simulink model "cll_zcs_ver_v"  (R2026b)
settings: Solver=ode23tb  StopTime=simlength  FixedStep=tc  MaxStep=tc  EnableMultiTasking=on
PostLoadFcn:
  | if any(exist('dsrtsu_mdlpostloadfcn', 'file') ~= 0), dsrtsu_mdlpostloadfcn('Execute', bdroot); end
InitFcn:
  | , if any(exist('rtifpga_mdlclblib', 'file') ~= 0), rtifpga_mdlclblib('Init', bdroot); end,
  | , if any(exist('dsmpb_private', 'file') ~= 0), dsmpb_private('dsmpb_mdlclblib', 'Init', bdroot); end,
values from neighbouring files (symbols this model uses):
  Adrso = eye(2) + Arso*ts    [init_zcs_model_ctrl.m]
  Adrsoh = eye(2) + Arsoh*ts    [init_zcs_model_ctrl.m]
  Crso = [1 0]    [init_zcs_model_ctrl.m]
  Crsoh = [1 0]    [init_zcs_model_ctrl.m]
  fres = 1/2/pi/sqrt(Cs*(Ls+L1sigma))    [init_zcs_model_ctrl.m]
  I_FS = Iout_dc_nom * margin_factor    (= 125)    [init_zcs_model_ctrl.m]
  Iout_ref_SI = 100*scale    (= 100)    [init_zcs_model_ctrl.m]
  k_h10_comp = -12    [init_zcs_model_ctrl.m]
  k_h12_comp = -12    [init_zcs_model_ctrl.m]
  k_h14_comp = -12    [init_zcs_model_ctrl.m]
  k_h2_comp = -12    [init_zcs_model_ctrl.m]
  k_h4_comp = -12    [init_zcs_model_ctrl.m]
  k_h6_comp = -12    [init_zcs_model_ctrl.m]
  k_h8_comp = -12    [init_zcs_model_ctrl.m]
  ki_i_zcs = 80    [init_zcs_model_ctrl.m]
  ki_v_zcs = 80    [init_zcs_model_ctrl.m]
  kp_i_zcs = 0.25    [init_zcs_model_ctrl.m]
  kp_v_zcs = 0.25    [init_zcs_model_ctrl.m]
  Ldrso = acker(Adrso',Crso',polesdrso)'    [init_zcs_model_ctrl.m]
  Ldrsoh = acker(Adrsoh',Crsoh',polesdrsoh)'    [init_zcs_model_ctrl.m]
  omega_grid_emu_nom = w_grid    (= 314.159265359)    [grid_emulator.m]
  omega_grid_nom = w_grid    (= 314.159265359)    [grid_emulator.m]
  pll_i1 = 80    [init_zcs_model_ctrl.m]
  pll_p = 1    [init_zcs_model_ctrl.m]
  q1kalman = ts/10    (= 1e-05)    [init_zcs_model_ctrl.m]
  q2kalman = ts/10    (= 1e-05)    [init_zcs_model_ctrl.m]
  Rkalman = 1/ts    (= 10000)    [init_zcs_model_ctrl.m]
  tc = 1e-7    (= 1e-07)    [init_zcs_model_ctrl.m]
  ts = 1e-4    (= 0.0001)    [init_zcs_model_ctrl.m]
  V_FS = Vout_dc_nom * margin_factor    (= 12.5)    [init_zcs_model_ctrl.m]
  V_phase_normalization_factor = Vgrid_phase_normalization_factor    [grid_emulator.m]
  Vgrid_phase_normalization_factor = Vphase2*sqrt(2)    [grid_emulator.m]
  vn_eta_pu = 0.05    [init_zcs_model_ctrl.m]
  vn_xi_pu = 0.05    [init_zcs_model_ctrl.m]
  Vout_dc_nom = 10    [init_zcs_model_ctrl.m]
  vp_xi_pu = 0.9    [init_zcs_model_ctrl.m]
undefined symbols (not defined in the file or in its folder): magnitude
libraries: fl_lib x55, nesl_utility x18, cstblocks_lti x7, single_phase_transformer_lib x1
(part 2 of 2)

== system cll_zcs_ver_v/vi_ctrl/sampling_v_filter1 ==
  in : Inport
  1/Ti3 : Gain  Gain=1/V_FS  OutDataTypeStr=double  SaturateOnIntegerOverflow=on  ParamDataTypeStr=Inherit: Same as input
  Saturation : Saturate  UpperLimit=1  LowerLimit=0  OutDataTypeStr=double
  Zero-Order Hold2 : ZeroOrderHold  SampleTime=ts
  out_pu : Outport
  wires:
  Zero-Order Hold2/1 -> out_pu/1
  1/Ti3/1 -> Saturation/1
  in/1 -> 1/Ti3/1
  Saturation/1 -> Zero-Order Hold2/1

== system cll_zcs_ver_v/vi_ctrl/sampling_v_filter2 ==
  in : Inport
  1/Ti3 : Gain  Gain=1/V_FS  OutDataTypeStr=double  SaturateOnIntegerOverflow=on  ParamDataTypeStr=Inherit: Same as input
  Saturation : Saturate  UpperLimit=1  LowerLimit=0  OutDataTypeStr=double
  Zero-Order Hold2 : ZeroOrderHold  SampleTime=ts
  out_pu : Outport
  wires:
  in/1 -> 1/Ti3/1
  1/Ti3/1 -> Saturation/1
  Zero-Order Hold2/1 -> out_pu/1
  Saturation/1 -> Zero-Order Hold2/1

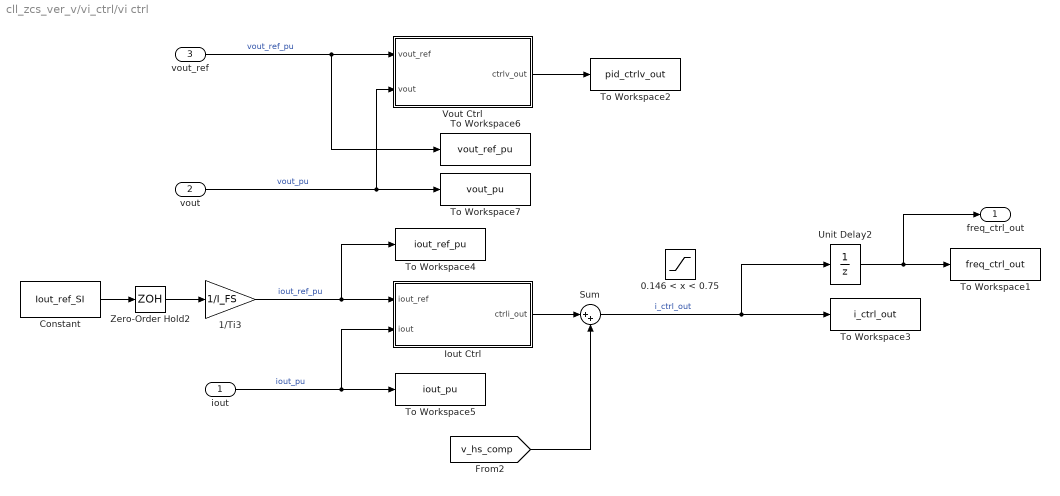
== system cll_zcs_ver_v/vi_ctrl/vi ctrl ==
  iout : Inport
  vout : Inport  Port=2
  vout_ref : Inport  Port=3
  0.146 < x < 0.75 : Saturate  UpperLimit=0.75  LowerLimit=0.146  OutDataTypeStr=double
  1/Ti3 : Gain  Gain=1/I_FS  OutDataTypeStr=double  SaturateOnIntegerOverflow=on  ParamDataTypeStr=Inherit: Same as input
  Constant : Constant  Value=Iout_ref_SI
  Iout Ctrl : Subsystem
  Sum : Sum  Inputs=|++
  To Workspace1 : ToWorkspace  VariableName=freq_ctrl_out  SampleTime=ts
      settings: MaxDataPoints=Ns
  To Workspace2 : ToWorkspace  VariableName=pid_ctrlv_out  SampleTime=ts
      settings: MaxDataPoints=Ns  Save2DSignal=2-D array (concatenate along first dimension)
  To Workspace3 : ToWorkspace  VariableName=i_ctrl_out  SampleTime=ts
      settings: MaxDataPoints=Ns  Save2DSignal=2-D array (concatenate along first dimension)
  To Workspace4 : ToWorkspace  VariableName=iout_ref_pu  SampleTime=ts
      settings: MaxDataPoints=Ns  Save2DSignal=2-D array (concatenate along first dimension)
  To Workspace5 : ToWorkspace  VariableName=iout_pu  SampleTime=ts
      settings: MaxDataPoints=Ns  Save2DSignal=2-D array (concatenate along first dimension)
  To Workspace6 : ToWorkspace  VariableName=vout_ref_pu  SampleTime=ts
      settings: MaxDataPoints=Ns  Save2DSignal=2-D array (concatenate along first dimension)
  To Workspace7 : ToWorkspace  VariableName=vout_pu  SampleTime=ts
      settings: MaxDataPoints=Ns  Save2DSignal=2-D array (concatenate along first dimension)
  Unit Delay2 : UnitDelay  SampleTime=ts
  Vout Ctrl : Subsystem
  Zero-Order Hold2 : ZeroOrderHold  SampleTime=ts
  freq_ctrl_out : Outport
  wires:
  Unit Delay2/1 -> To Workspace1/1, freq_ctrl_out/1
  iout/1 -> To Workspace5/1, Iout Ctrl/2(iout)  "iout_pu"
  vout_ref/1 -> To Workspace6/1, Vout Ctrl/1(vout_ref)  "vout_ref_pu"
  vout/1 -> Vout Ctrl/2(vout), To Workspace7/1  "vout_pu"
  Vout Ctrl/1(ctrlv_out) -> To Workspace2/1
  Constant/1 -> Zero-Order Hold2/1
  1/Ti3/1 -> To Workspace4/1, Iout Ctrl/1(iout_ref)  "iout_ref_pu"
  Iout Ctrl/1(ctrli_out) -> Sum/1
  Zero-Order Hold2/1 -> 1/Ti3/1
  Sum/1 -> Unit Delay2/1, To Workspace3/1  "i_ctrl_out"
  [v_hs_comp] -> Sum/2

== system cll_zcs_ver_v/PLL/pll_stageA/mormalization_and_transformation ==
  ug_a : Inport
  ug_b : Inport  Port=2
  ug_c : Inport  Port=3
  Gain1 : Gain  Gain=1/Vgrid_phase_normalization_factor
  Gain2 : Gain  Gain=1/Vgrid_phase_normalization_factor
  Gain3 : Gain  Gain=1/Vgrid_phase_normalization_factor
  Zero-Order Hold : ZeroOrderHold  SampleTime=ts
  Zero-Order Hold1 : ZeroOrderHold  SampleTime=ts
  Zero-Order Hold2 : ZeroOrderHold  SampleTime=ts
  abc2alphabeta : MATLAB Function  TreatAsAtomicUnit=on
  ug_alpha : Outport  VectorParamsAs1DForOutWhenUnconnected=off
  ug_beta : Outport  Port=2  VectorParamsAs1DForOutWhenUnconnected=off
  wires:
  abc2alphabeta/1(alpha) -> ug_alpha/1  "u_grid_alpha"
  abc2alphabeta/2(beta) -> ug_beta/1  "u_grid_beta"
  Gain3/1 -> abc2alphabeta/3(c)
  Gain2/1 -> abc2alphabeta/2(b)
  Gain1/1 -> abc2alphabeta/1(a)
  Zero-Order Hold2/1 -> Gain3/1
  Zero-Order Hold1/1 -> Gain2/1
  Zero-Order Hold/1 -> Gain1/1
  ug_b/1 -> Zero-Order Hold1/1
  ug_c/1 -> Zero-Order Hold2/1
  ug_a/1 -> Zero-Order Hold/1

== system cll_zcs_ver_v/PLL/pll_stageA/sequences ==
  u_grid_alpha : Inport
  u_grid_beta : Inport  Port=2
  phase_angle : Inport  Port=3
  ddsrf : Subsystem
  u_grid_pos_xi : Outport
  u_grid_pos_eta : Outport  Port=2
  wires:
  phase_angle/1 -> ddsrf/3(phase_angle)  "phase_angle"
  u_grid_beta/1 -> ddsrf/2(u_grid_beta)  "u_grid_beta"
  u_grid_alpha/1 -> ddsrf/1(u_grid_alpha)  "u_grid_alpha"
  ddsrf/2(u_grid_pos_eta) -> u_grid_pos_eta/1  "u_grid_pos_eta"
  ddsrf/1(u_grid_pos_xi) -> u_grid_pos_xi/1  "u_grid_pos_xi"

== system cll_zcs_ver_v/PLL/pll_stageB/double_integrator_observer ==
  theta : Inport
  Gain : Gain  Gain=Ldrso  Multiplication=Matrix(K*u)
  Gain1 : Gain  Gain=Adrso  Multiplication=Matrix(K*u)
  Gain2 : Gain  Gain=Crso  Multiplication=Matrix(K*u)
  Selector : Selector  InputPortWidth=2  IndexOptions=Index vector (dialog)  Indices=2  OutputSizes=1  RuntimeRangeChecks=off
  Sum : Sum  Inputs=-+|
  Sum1 : Sum  Inputs=|++
  Unit Delay : UnitDelay  SampleTime=ts
  Zero-Order Hold : ZeroOrderHold  SampleTime=ts
  bounder1 : MATLAB Function  TreatAsAtomicUnit=on  SystemSampleTime=ts
  bounder2 : MATLAB Function  TreatAsAtomicUnit=on  SystemSampleTime=ts
  omega_hat : Outport
  wires:
  bounder2/1(y) -> Sum/1  "theta_hat_bounded"
  bounder1/1(y) -> Gain/1  "e_bounded"
  Zero-Order Hold/1 -> Sum/2  "theta_dsp"
  theta/1 -> Zero-Order Hold/1  "theta"
  Unit Delay/1 -> Gain2/1, Selector/1, Gain1/1
  Sum/1 -> bounder1/1(u)  "e"
  Sum1/1 -> Unit Delay/1
  Gain1/1 -> Sum1/2
  Gain2/1 -> bounder2/1(u)  "theta_hat"
  Selector/1 -> omega_hat/1
  Gain/1 -> Sum1/1

== system cll_zcs_ver_v/cll_zcs/HBridge/switch_1 ==
  g : Inport
  D : fl_lib/Electrical/Electrical Elements/Diode  Vf=0.6 V  Ron=1e-3 Ohm  Goff=1e-8 1/Ohm  i_specify=off  i_priority=None  i=0 A  i_nominal_specify=off  i_nominal_value=1  i_nominal_unit=A  v_specify=off  v_priority=None  v=0 V  v_nominal_specify=off  v_nominal_value=1  v_nominal_unit=V
  Q : fl_lib/Electrical/Electrical Elements/Switch  R_closed=1e-3 Ohm  G_open=1e-8 1/Ohm  Threshold=0.5  i_specify=off  i_priority=None  i=0 A  i_nominal_specify=off  i_nominal_value=1  i_nominal_unit=A  v_specify=off  v_priority=None  v=0 V  v_nominal_specify=off  v_nominal_value=1  v_nominal_unit=V
  RCsnubber : fl_lib/Electrical/Electrical Elements/Capacitor  c=Csnubber F  r=Rsnubber Ohm  g=0 1/Ohm  i_specify=off  i_priority=None  i=0 A  i_nominal_specify=off  i_nominal_value=1  i_nominal_unit=A  v_specify=off  v_priority=None  v=0 V  v_nominal_specify=off  v_nominal_value=1  v_nominal_unit=V  vc_specify=off  vc_priority=High  vc=0 V  vc_nominal_specify=off  vc_nominal_value=1  vc_nominal_unit=V
  Simulink-PS Converter : nesl_utility/Simulink-PS Converter  PhysicalDomain=network_engine_domain  SubClassName=ps_input  LeftPortType=input  RightPortType=output  PseudoPeriodic=off  Frequencies=[]  NoiseDistribution=none  NoiseParameters=[]  Unit=1  AffineConversion=off  FilteringAndDerivatives=provide  SimscapeFilterOrder=1  InputFilterTimeConstant=0.001  UdotUserProvided=0
  d : PMIOPort  Side=Left
  s : PMIOPort  Port=2  Side=Right
  wires:
  g/1 -> Simulink-PS Converter/1
  connections:
  Q/RConn2 -- D/LConn1 -- s/RConn1 -- RCsnubber/RConn1
  Simulink-PS Converter/RConn1 -- Q/RConn1
  Q/LConn1 -- RCsnubber/LConn1 -- d/RConn1 -- D/RConn1

== system cll_zcs_ver_v/cll_zcs/HBridge/switch_2 ==
  g : Inport
  D : fl_lib/Electrical/Electrical Elements/Diode  Vf=0.6 V  Ron=1e-3 Ohm  Goff=1e-8 1/Ohm  i_specify=off  i_priority=None  i=0 A  i_nominal_specify=off  i_nominal_value=1  i_nominal_unit=A  v_specify=off  v_priority=None  v=0 V  v_nominal_specify=off  v_nominal_value=1  v_nominal_unit=V
  Q : fl_lib/Electrical/Electrical Elements/Switch  R_closed=1e-3 Ohm  G_open=1e-8 1/Ohm  Threshold=0.5  i_specify=off  i_priority=None  i=0 A  i_nominal_specify=off  i_nominal_value=1  i_nominal_unit=A  v_specify=off  v_priority=None  v=0 V  v_nominal_specify=off  v_nominal_value=1  v_nominal_unit=V
  RCsnubber : fl_lib/Electrical/Electrical Elements/Capacitor  c=Csnubber F  r=Rsnubber Ohm  g=0 1/Ohm  i_specify=off  i_priority=None  i=0 A  i_nominal_specify=off  i_nominal_value=1  i_nominal_unit=A  v_specify=off  v_priority=None  v=0 V  v_nominal_specify=off  v_nominal_value=1  v_nominal_unit=V  vc_specify=off  vc_priority=High  vc=0 V  vc_nominal_specify=off  vc_nominal_value=1  vc_nominal_unit=V
  Simulink-PS Converter : nesl_utility/Simulink-PS Converter  PhysicalDomain=network_engine_domain  SubClassName=ps_input  LeftPortType=input  RightPortType=output  PseudoPeriodic=off  Frequencies=[]  NoiseDistribution=none  NoiseParameters=[]  Unit=1  AffineConversion=off  FilteringAndDerivatives=provide  SimscapeFilterOrder=1  InputFilterTimeConstant=0.001  UdotUserProvided=0
  d : PMIOPort  Side=Left
  s : PMIOPort  Port=2  Side=Right
  wires:
  g/1 -> Simulink-PS Converter/1
  connections:
  d/RConn1 -- RCsnubber/LConn1 -- Q/LConn1 -- D/RConn1
  Simulink-PS Converter/RConn1 -- Q/RConn1
  s/RConn1 -- RCsnubber/RConn1 -- D/LConn1 -- Q/RConn2

== system cll_zcs_ver_v/grid/grid_emulator/grid_emulator ==
  phase_gen : Subsystem
  voltage_reference : Subsystem
  voltage_source : Subsystem
  Vma : Outport
  Vmb : Outport  Port=2
  Vmc : Outport  Port=3
  wires:
  phase_gen/1(grid_emu_phase) -> voltage_reference/1(grid_emu_phase)  "grid_emu_phase"
  voltage_source/2(vn_xi) -> voltage_reference/3(Vxi_n)
  voltage_source/1(vp_xi) -> voltage_reference/2(Vxi_p)
  voltage_source/3(vn_eta) -> voltage_reference/4(Veta_n)
  voltage_reference/3(V3_ref) -> Vmc/1
  voltage_reference/1(V1_ref) -> Vma/1
  voltage_reference/2(V2_ref) -> Vmb/1

== system cll_zcs_ver_v/hs_compensation/magnitude_100Hz_harmonic_detection/double_integrator_observer ==
  theta : Inport
  Gain : Gain  Gain=Ldrsoh  Multiplication=Matrix(K*u)
  Gain1 : Gain  Gain=Adrsoh  Multiplication=Matrix(K*u)
  Gain2 : Gain  Gain=Crsoh  Multiplication=Matrix(K*u)
  Selector : Selector  InputPortWidth=2  IndexOptions=Index vector (dialog)  Indices=2  OutputSizes=1  RuntimeRangeChecks=off
  Sum : Sum  Inputs=-+|
  Sum1 : Sum  Inputs=|++
  Unit Delay : UnitDelay  SampleTime=ts
  Zero-Order Hold : ZeroOrderHold  SampleTime=ts
  bounder1 : MATLAB Function  TreatAsAtomicUnit=on  SystemSampleTime=ts
  bounder2 : MATLAB Function  TreatAsAtomicUnit=on  SystemSampleTime=ts
  omega_hat : Outport
  theta_hat : Outport  Port=2
  wires:
  Gain/1 -> Sum1/1
  Selector/1 -> omega_hat/1
  Gain2/1 -> bounder2/1(u)  "theta_hat"
  Gain1/1 -> Sum1/2
  Sum1/1 -> Unit Delay/1
  Sum/1 -> bounder1/1(u)  "e"
  Unit Delay/1 -> Gain1/1, Selector/1, Gain2/1
  theta/1 -> Zero-Order Hold/1  "theta"
  Zero-Order Hold/1 -> Sum/2  "theta_dsp"
  bounder1/1(y) -> Gain/1  "e_bounded"
  bounder2/1(y) -> theta_hat/1, Sum/1  "theta_hat_bounded"

== system cll_zcs_ver_v/hs_compensation/magnitude_100Hz_harmonic_detection/magnitude ==
  alpha : Inport
  beta : Inport  Port=2
  Math Function : Math  Operator=magnitude^2
  Math Function1 : Math  Operator=magnitude^2
  Sqrt : Sqrt
  Sum : Sum  Inputs=|++
  a : Outport
  wires:
  Sqrt/1 -> a/1
  Sum/1 -> Sqrt/1
  Math Function1/1 -> Sum/2
  Math Function/1 -> Sum/1
  beta/1 -> Math Function1/1
  alpha/1 -> Math Function/1

== system cll_zcs_ver_v/hs_compensation/magnitude_200Hz_harmonic_detection/double_integrator_observer ==
  theta : Inport
  Gain : Gain  Gain=Ldrsoh  Multiplication=Matrix(K*u)
  Gain1 : Gain  Gain=Adrsoh  Multiplication=Matrix(K*u)
  Gain2 : Gain  Gain=Crsoh  Multiplication=Matrix(K*u)
  Selector : Selector  InputPortWidth=2  IndexOptions=Index vector (dialog)  Indices=2  OutputSizes=1  RuntimeRangeChecks=off
  Sum : Sum  Inputs=-+|
  Sum1 : Sum  Inputs=|++
  Unit Delay : UnitDelay  SampleTime=ts
  Zero-Order Hold : ZeroOrderHold  SampleTime=ts
  bounder1 : MATLAB Function  TreatAsAtomicUnit=on  SystemSampleTime=ts
  bounder2 : MATLAB Function  TreatAsAtomicUnit=on  SystemSampleTime=ts
  omega_hat : Outport
  theta_hat : Outport  Port=2
  wires:
  Gain/1 -> Sum1/1
  Selector/1 -> omega_hat/1
  Gain2/1 -> bounder2/1(u)  "theta_hat"
  Gain1/1 -> Sum1/2
  Sum1/1 -> Unit Delay/1
  Sum/1 -> bounder1/1(u)  "e"
  Unit Delay/1 -> Gain1/1, Selector/1, Gain2/1
  theta/1 -> Zero-Order Hold/1  "theta"
  Zero-Order Hold/1 -> Sum/2  "theta_dsp"
  bounder1/1(y) -> Gain/1  "e_bounded"
  bounder2/1(y) -> theta_hat/1, Sum/1  "theta_hat_bounded"

== system cll_zcs_ver_v/hs_compensation/magnitude_200Hz_harmonic_detection/magnitude ==
  alpha : Inport
  beta : Inport  Port=2
  Math Function : Math  Operator=magnitude^2
  Math Function1 : Math  Operator=magnitude^2
  Sqrt : Sqrt
  Sum : Sum  Inputs=|++
  a : Outport
  wires:
  alpha/1 -> Math Function/1
  beta/1 -> Math Function1/1
  Math Function/1 -> Sum/1
  Math Function1/1 -> Sum/2
  Sum/1 -> Sqrt/1
  Sqrt/1 -> a/1

== system cll_zcs_ver_v/hs_compensation/magnitude_300Hz_harmonic_detection/double_integrator_observer ==
  theta : Inport
  Gain : Gain  Gain=Ldrsoh  Multiplication=Matrix(K*u)
  Gain1 : Gain  Gain=Adrsoh  Multiplication=Matrix(K*u)
  Gain2 : Gain  Gain=Crsoh  Multiplication=Matrix(K*u)
  Selector : Selector  InputPortWidth=2  IndexOptions=Index vector (dialog)  Indices=2  OutputSizes=1  RuntimeRangeChecks=off
  Sum : Sum  Inputs=-+|
  Sum1 : Sum  Inputs=|++
  Unit Delay : UnitDelay  SampleTime=ts
  Zero-Order Hold : ZeroOrderHold  SampleTime=ts
  bounder1 : MATLAB Function  TreatAsAtomicUnit=on  SystemSampleTime=ts
  bounder2 : MATLAB Function  TreatAsAtomicUnit=on  SystemSampleTime=ts
  omega_hat : Outport
  theta_hat : Outport  Port=2
  wires:
  Gain/1 -> Sum1/1
  Selector/1 -> omega_hat/1
  Gain2/1 -> bounder2/1(u)  "theta_hat"
  Gain1/1 -> Sum1/2
  Sum1/1 -> Unit Delay/1
  Sum/1 -> bounder1/1(u)  "e"
  Unit Delay/1 -> Gain1/1, Selector/1, Gain2/1
  theta/1 -> Zero-Order Hold/1  "theta"
  Zero-Order Hold/1 -> Sum/2  "theta_dsp"
  bounder1/1(y) -> Gain/1  "e_bounded"
  bounder2/1(y) -> theta_hat/1, Sum/1  "theta_hat_bounded"

== system cll_zcs_ver_v/hs_compensation/magnitude_300Hz_harmonic_detection/magnitude ==
  alpha : Inport
  beta : Inport  Port=2
  Math Function : Math  Operator=magnitude^2
  Math Function1 : Math  Operator=magnitude^2
  Sqrt : Sqrt
  Sum : Sum  Inputs=|++
  a : Outport
  wires:
  alpha/1 -> Math Function/1
  beta/1 -> Math Function1/1
  Math Function/1 -> Sum/1
  Math Function1/1 -> Sum/2
  Sum/1 -> Sqrt/1
  Sqrt/1 -> a/1

== system cll_zcs_ver_v/hs_compensation/magnitude_400Hz_harmonic_detection/double_integrator_observer ==
  theta : Inport
  Gain : Gain  Gain=Ldrsoh  Multiplication=Matrix(K*u)
  Gain1 : Gain  Gain=Adrsoh  Multiplication=Matrix(K*u)
  Gain2 : Gain  Gain=Crsoh  Multiplication=Matrix(K*u)
  Selector : Selector  InputPortWidth=2  IndexOptions=Index vector (dialog)  Indices=2  OutputSizes=1  RuntimeRangeChecks=off
  Sum : Sum  Inputs=-+|
  Sum1 : Sum  Inputs=|++
  Unit Delay : UnitDelay  SampleTime=ts
  Zero-Order Hold : ZeroOrderHold  SampleTime=ts
  bounder1 : MATLAB Function  TreatAsAtomicUnit=on  SystemSampleTime=ts
  bounder2 : MATLAB Function  TreatAsAtomicUnit=on  SystemSampleTime=ts
  omega_hat : Outport
  theta_hat : Outport  Port=2
  wires:
  Gain/1 -> Sum1/1
  Selector/1 -> omega_hat/1
  Gain2/1 -> bounder2/1(u)  "theta_hat"
  Gain1/1 -> Sum1/2
  Sum1/1 -> Unit Delay/1
  Sum/1 -> bounder1/1(u)  "e"
  Unit Delay/1 -> Gain1/1, Selector/1, Gain2/1
  theta/1 -> Zero-Order Hold/1  "theta"
  Zero-Order Hold/1 -> Sum/2  "theta_dsp"
  bounder1/1(y) -> Gain/1  "e_bounded"
  bounder2/1(y) -> theta_hat/1, Sum/1  "theta_hat_bounded"

== system cll_zcs_ver_v/hs_compensation/magnitude_400Hz_harmonic_detection/magnitude ==
  alpha : Inport
  beta : Inport  Port=2
  Math Function : Math  Operator=magnitude^2
  Math Function1 : Math  Operator=magnitude^2
  Sqrt : Sqrt
  Sum : Sum  Inputs=|++
  a : Outport
  wires:
  alpha/1 -> Math Function/1
  beta/1 -> Math Function1/1
  Math Function/1 -> Sum/1
  Math Function1/1 -> Sum/2
  Sum/1 -> Sqrt/1
  Sqrt/1 -> a/1

== system cll_zcs_ver_v/hs_compensation/magnitude_500Hz_harmonic_detection/double_integrator_observer ==
  theta : Inport
  Gain : Gain  Gain=Ldrsoh  Multiplication=Matrix(K*u)
  Gain1 : Gain  Gain=Adrsoh  Multiplication=Matrix(K*u)
  Gain2 : Gain  Gain=Crsoh  Multiplication=Matrix(K*u)
  Selector : Selector  InputPortWidth=2  IndexOptions=Index vector (dialog)  Indices=2  OutputSizes=1  RuntimeRangeChecks=off
  Sum : Sum  Inputs=-+|
  Sum1 : Sum  Inputs=|++
  Unit Delay : UnitDelay  SampleTime=ts
  Zero-Order Hold : ZeroOrderHold  SampleTime=ts
  bounder1 : MATLAB Function  TreatAsAtomicUnit=on  SystemSampleTime=ts
  bounder2 : MATLAB Function  TreatAsAtomicUnit=on  SystemSampleTime=ts
  omega_hat : Outport
  theta_hat : Outport  Port=2
  wires:
  Gain/1 -> Sum1/1
  Selector/1 -> omega_hat/1
  Gain2/1 -> bounder2/1(u)  "theta_hat"
  Gain1/1 -> Sum1/2
  Sum1/1 -> Unit Delay/1
  Sum/1 -> bounder1/1(u)  "e"
  Unit Delay/1 -> Gain1/1, Selector/1, Gain2/1
  theta/1 -> Zero-Order Hold/1  "theta"
  Zero-Order Hold/1 -> Sum/2  "theta_dsp"
  bounder1/1(y) -> Gain/1  "e_bounded"
  bounder2/1(y) -> theta_hat/1, Sum/1  "theta_hat_bounded"

== system cll_zcs_ver_v/hs_compensation/magnitude_500Hz_harmonic_detection/magnitude ==
  alpha : Inport
  beta : Inport  Port=2
  Math Function : Math  Operator=magnitude^2
  Math Function1 : Math  Operator=magnitude^2
  Sqrt : Sqrt
  Sum : Sum  Inputs=|++
  a : Outport
  wires:
  Sqrt/1 -> a/1
  Sum/1 -> Sqrt/1
  Math Function1/1 -> Sum/2
  Math Function/1 -> Sum/1
  beta/1 -> Math Function1/1
  alpha/1 -> Math Function/1

== system cll_zcs_ver_v/hs_compensation/magnitude_600Hz_harmonic_detection/double_integrator_observer ==
  theta : Inport
  Gain : Gain  Gain=Ldrsoh  Multiplication=Matrix(K*u)
  Gain1 : Gain  Gain=Adrsoh  Multiplication=Matrix(K*u)
  Gain2 : Gain  Gain=Crsoh  Multiplication=Matrix(K*u)
  Selector : Selector  InputPortWidth=2  IndexOptions=Index vector (dialog)  Indices=2  OutputSizes=1  RuntimeRangeChecks=off
  Sum : Sum  Inputs=-+|
  Sum1 : Sum  Inputs=|++
  Unit Delay : UnitDelay  SampleTime=ts
  Zero-Order Hold : ZeroOrderHold  SampleTime=ts
  bounder1 : MATLAB Function  TreatAsAtomicUnit=on  SystemSampleTime=ts
  bounder2 : MATLAB Function  TreatAsAtomicUnit=on  SystemSampleTime=ts
  omega_hat : Outport
  theta_hat : Outport  Port=2
  wires:
  Gain/1 -> Sum1/1
  Selector/1 -> omega_hat/1
  Gain2/1 -> bounder2/1(u)  "theta_hat"
  Gain1/1 -> Sum1/2
  Sum1/1 -> Unit Delay/1
  Sum/1 -> bounder1/1(u)  "e"
  Unit Delay/1 -> Gain1/1, Selector/1, Gain2/1
  theta/1 -> Zero-Order Hold/1  "theta"
  Zero-Order Hold/1 -> Sum/2  "theta_dsp"
  bounder1/1(y) -> Gain/1  "e_bounded"
  bounder2/1(y) -> theta_hat/1, Sum/1  "theta_hat_bounded"

== system cll_zcs_ver_v/hs_compensation/magnitude_600Hz_harmonic_detection/magnitude ==
  alpha : Inport
  beta : Inport  Port=2
  Math Function : Math  Operator=magnitude^2
  Math Function1 : Math  Operator=magnitude^2
  Sqrt : Sqrt
  Sum : Sum  Inputs=|++
  a : Outport
  wires:
  Sqrt/1 -> a/1
  Sum/1 -> Sqrt/1
  Math Function1/1 -> Sum/2
  Math Function/1 -> Sum/1
  beta/1 -> Math Function1/1
  alpha/1 -> Math Function/1

== system cll_zcs_ver_v/hs_compensation/magnitude_700Hz_harmonic_detection/double_integrator_observer ==
  theta : Inport
  Gain : Gain  Gain=Ldrsoh  Multiplication=Matrix(K*u)
  Gain1 : Gain  Gain=Adrsoh  Multiplication=Matrix(K*u)
  Gain2 : Gain  Gain=Crsoh  Multiplication=Matrix(K*u)
  Selector : Selector  InputPortWidth=2  IndexOptions=Index vector (dialog)  Indices=2  OutputSizes=1  RuntimeRangeChecks=off
  Sum : Sum  Inputs=-+|
  Sum1 : Sum  Inputs=|++
  Unit Delay : UnitDelay  SampleTime=ts
  Zero-Order Hold : ZeroOrderHold  SampleTime=ts
  bounder1 : MATLAB Function  TreatAsAtomicUnit=on  SystemSampleTime=ts
  bounder2 : MATLAB Function  TreatAsAtomicUnit=on  SystemSampleTime=ts
  omega_hat : Outport
  theta_hat : Outport  Port=2
  wires:
  Gain/1 -> Sum1/1
  Selector/1 -> omega_hat/1
  Gain2/1 -> bounder2/1(u)  "theta_hat"
  Gain1/1 -> Sum1/2
  Sum1/1 -> Unit Delay/1
  Sum/1 -> bounder1/1(u)  "e"
  Unit Delay/1 -> Gain1/1, Selector/1, Gain2/1
  theta/1 -> Zero-Order Hold/1  "theta"
  Zero-Order Hold/1 -> Sum/2  "theta_dsp"
  bounder1/1(y) -> Gain/1  "e_bounded"
  bounder2/1(y) -> theta_hat/1, Sum/1  "theta_hat_bounded"

== system cll_zcs_ver_v/hs_compensation/magnitude_700Hz_harmonic_detection/magnitude ==
  alpha : Inport
  beta : Inport  Port=2
  Math Function : Math  Operator=magnitude^2
  Math Function1 : Math  Operator=magnitude^2
  Sqrt : Sqrt
  Sum : Sum  Inputs=|++
  a : Outport
  wires:
  alpha/1 -> Math Function/1
  beta/1 -> Math Function1/1
  Math Function/1 -> Sum/1
  Math Function1/1 -> Sum/2
  Sum/1 -> Sqrt/1
  Sqrt/1 -> a/1

== system cll_zcs_ver_v/vi_ctrl/references/voltage_reference ==
  Constant1 : Constant  Value=Vout_dc_nom
  To Workspace2 : ToWorkspace  VariableName=vout_ref  SampleTime=ts
      settings: MaxDataPoints=Ns
  vout_ref : Outport
  wires:
  Constant1/1 -> To Workspace2/1, vout_ref/1

== system cll_zcs_ver_v/vi_ctrl/vi ctrl/Iout Ctrl ==
  iout_ref : Inport
  iout : Inport  Port=2
  Sum2 : Sum  Inputs=+-  OutDataTypeStr=double  AccumDataTypeStr=double  SaturateOnIntegerOverflow=on
  iout_ctrl : Subsystem
  ctrli_out : Outport
  wires:
  iout_ctrl/1(ctrli_out) -> ctrli_out/1
  iout/1 -> Sum2/2
  iout_ref/1 -> Sum2/1
  Sum2/1 -> iout_ctrl/1(i_tilde)

== system cll_zcs_ver_v/vi_ctrl/vi ctrl/Vout Ctrl ==
  vout_ref : Inport
  vout : Inport  Port=2
  Sum2 : Sum  Inputs=+-  OutDataTypeStr=double  AccumDataTypeStr=double  SaturateOnIntegerOverflow=on
  vout_ctrl : Subsystem
  ctrlv_out : Outport
  wires:
  vout_ref/1 -> Sum2/1
  vout/1 -> Sum2/2
  vout_ctrl/1(ctrlv_out) -> ctrlv_out/1
  Sum2/1 -> vout_ctrl/1(ixi_tilde)

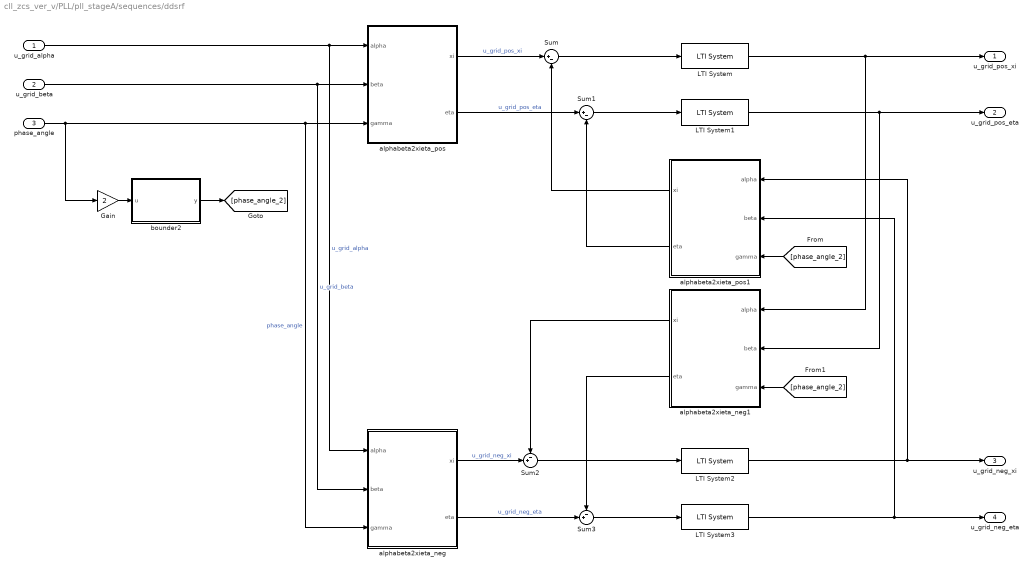
== system cll_zcs_ver_v/PLL/pll_stageA/sequences/ddsrf ==
  u_grid_alpha : Inport
  u_grid_beta : Inport  Port=2
  phase_angle : Inport  Port=3
  Gain : Gain  Gain=2
  LTI System{,1..3} (4 alike) : cstblocks_lti/LTI System  sys=ddsrf_fd  IC=[]  PadeOrder=0
  Sum : Sum  Inputs=|+-
  Sum1 : Sum  Inputs=|+-
  Sum2 : Sum  Inputs=-+|
  Sum3 : Sum  Inputs=-+|
  alphabeta2xieta_neg : MATLAB Function  TreatAsAtomicUnit=on
  alphabeta2xieta_neg1 : MATLAB Function  TreatAsAtomicUnit=on
  alphabeta2xieta_pos : MATLAB Function  TreatAsAtomicUnit=on
  alphabeta2xieta_pos1 : MATLAB Function  TreatAsAtomicUnit=on
  bounder2 : MATLAB Function  TreatAsAtomicUnit=on  SystemSampleTime=ts
  u_grid_pos_xi : Outport
  u_grid_pos_eta : Outport  Port=2
  u_grid_neg_xi : Outport  Port=3
  u_grid_neg_eta : Outport  Port=4
  wires:
  phase_angle/1 -> alphabeta2xieta_pos/3(gamma), alphabeta2xieta_neg/3(gamma), Gain/1  "phase_angle"
  u_grid_beta/1 -> alphabeta2xieta_pos/2(beta), alphabeta2xieta_neg/2(beta)  "u_grid_beta"
  u_grid_alpha/1 -> alphabeta2xieta_pos/1(alpha), alphabeta2xieta_neg/1(alpha)  "u_grid_alpha"
  alphabeta2xieta_pos/1(xi) -> Sum/1  "u_grid_pos_xi"
  Sum/1 -> LTI System/1
  alphabeta2xieta_pos/2(eta) -> Sum1/1  "u_grid_pos_eta"
  Sum1/1 -> LTI System1/1
  alphabeta2xieta_neg/1(xi) -> Sum2/2  "u_grid_neg_xi"
  Sum2/1 -> LTI System2/1
  Sum3/1 -> LTI System3/1
  alphabeta2xieta_neg/2(eta) -> Sum3/2  "u_grid_neg_eta"
  Gain/1 -> bounder2/1(u)
  LTI System/1 -> alphabeta2xieta_neg1/1(alpha), u_grid_pos_xi/1
  LTI System1/1 -> alphabeta2xieta_neg1/2(beta), u_grid_pos_eta/1
  LTI System2/1 -> u_grid_neg_xi/1, alphabeta2xieta_pos1/1(alpha)
  LTI System3/1 -> u_grid_neg_eta/1, alphabeta2xieta_pos1/2(beta)
  bounder2/1(y) -> [phase_angle_2]
  [phase_angle_2] -> alphabeta2xieta_pos1/3(gamma)
  [phase_angle_2] -> alphabeta2xieta_neg1/3(gamma)
  alphabeta2xieta_pos1/1(xi) -> Sum/2
  alphabeta2xieta_pos1/2(eta) -> Sum1/2
  alphabeta2xieta_neg1/1(xi) -> Sum2/1
  alphabeta2xieta_neg1/2(eta) -> Sum3/1

== system cll_zcs_ver_v/grid/grid_emulator/grid_emulator/phase_gen ==
  Constant4 : Constant  Value=omega_grid_emu_nom
  Integrator : Integrator
  To Workspace7 : ToWorkspace  VariableName=grid_emu_phase  SampleTime=ts
      settings: MaxDataPoints=Ns
  bounder1 : MATLAB Function  TreatAsAtomicUnit=on  SystemSampleTime=ts
  grid_emu_phase : Outport  VectorParamsAs1DForOutWhenUnconnected=off
  wires:
  bounder1/1(y) -> To Workspace7/1, grid_emu_phase/1  "grid_emu_phase"
  Constant4/1 -> Integrator/1
  Integrator/1 -> bounder1/1(u)

== system cll_zcs_ver_v/grid/grid_emulator/grid_emulator/voltage_reference ==
  grid_emu_phase : Inport
  Vxi_p : Inport  Port=2
  Vxi_n : Inport  Port=3
  Veta_n : Inport  Port=4
  Constant2 : Constant  Value=0
  Sum1 : Sum  Inputs=|++
  Sum4 : Sum  Inputs=|++
  alphabeta2abc : MATLAB Function  TreatAsAtomicUnit=on
  xieta2alphabeta_neg : MATLAB Function  TreatAsAtomicUnit=on
  xieta2alphabeta_pos : MATLAB Function  TreatAsAtomicUnit=on
  V1_ref : Outport  VectorParamsAs1DForOutWhenUnconnected=off
  V2_ref : Outport  Port=2  VectorParamsAs1DForOutWhenUnconnected=off
  V3_ref : Outport  Port=3  VectorParamsAs1DForOutWhenUnconnected=off
  wires:
  xieta2alphabeta_pos/1(alpha) -> Sum1/1
  Sum1/1 -> alphabeta2abc/1(alpha)
  xieta2alphabeta_pos/2(beta) -> Sum4/1
  Sum4/1 -> alphabeta2abc/2(beta)
  xieta2alphabeta_neg/1(alpha) -> Sum1/2
  xieta2alphabeta_neg/2(beta) -> Sum4/2
  alphabeta2abc/1(a) -> V1_ref/1
  alphabeta2abc/2(b) -> V2_ref/1
  alphabeta2abc/3(c) -> V3_ref/1
  grid_emu_phase/1 -> xieta2alphabeta_neg/3(gamma), xieta2alphabeta_pos/3(gamma)
  Vxi_p/1 -> xieta2alphabeta_pos/1(xi)
  Constant2/1 -> xieta2alphabeta_pos/2(eta)
  Vxi_n/1 -> xieta2alphabeta_neg/1(xi)
  Veta_n/1 -> xieta2alphabeta_neg/2(eta)

== system cll_zcs_ver_v/grid/grid_emulator/grid_emulator/voltage_source ==
  Constant : Constant  Value=vp_xi_pu
  Constant1 : Constant  Value=vn_xi_pu
  Constant2 : Constant  Value=vn_eta_pu
  Gain1 : Gain  Gain=V_phase_normalization_factor
  Gain7 : Gain  Gain=V_phase_normalization_factor
  Gain8 : Gain  Gain=V_phase_normalization_factor
  LTI System : cstblocks_lti/LTI System  sys=LVRT_flt_ss_c  IC=[]  PadeOrder=0
  LTI System1 : cstblocks_lti/LTI System  sys=LVRT_flt_ss_c  IC=[]  PadeOrder=0
  LTI System2 : cstblocks_lti/LTI System  sys=LVRT_flt_ss_c  IC=[]  PadeOrder=0
  vp_xi : Outport  VectorParamsAs1DForOutWhenUnconnected=off
  vn_xi : Outport  Port=2  VectorParamsAs1DForOutWhenUnconnected=off
  vn_eta : Outport  Port=3  VectorParamsAs1DForOutWhenUnconnected=off
  wires:
  Constant1/1 -> LTI System1/1
  LTI System/1 -> Gain7/1
  LTI System1/1 -> Gain8/1
  Constant/1 -> LTI System/1
  Gain7/1 -> vp_xi/1
  Gain8/1 -> vn_xi/1
  Gain1/1 -> vn_eta/1
  LTI System2/1 -> Gain1/1
  Constant2/1 -> LTI System2/1

== system cll_zcs_ver_v/vi_ctrl/vi ctrl/Iout Ctrl/iout_ctrl ==
  i_tilde : Inport
  0.146 < x < 0.6 : Saturate  UpperLimit=0.6  LowerLimit=0.146  OutDataTypeStr=double
  1/Ti : Gain  Gain=kp_i_zcs  ParamDataTypeStr=double  OutDataTypeStr=double  SaturateOnIntegerOverflow=on
  Sum1 : Sum  Inputs=+++  SaturateOnIntegerOverflow=on
  Sum4 : Sum  Inputs=-+  SaturateOnIntegerOverflow=on
  Unit Delay4 : UnitDelay  SampleTime=ts
  kp2 : Gain  Gain=ki_i_zcs*ts  ParamDataTypeStr=double  OutDataTypeStr=double  SaturateOnIntegerOverflow=on
  ctrli_out : Outport
  wires:
  i_tilde/1 -> kp2/1, 1/Ti/1
  Sum1/1 -> 0.146 < x < 0.6/1
  kp2/1 -> Sum1/2
  1/Ti/1 -> Sum1/1, Sum4/1
  Sum4/1 -> Unit Delay4/1
  Unit Delay4/1 -> Sum1/3
  0.146 < x < 0.6/1 -> Sum4/2, ctrli_out/1  "i_ctrl_out"

== system cll_zcs_ver_v/vi_ctrl/vi ctrl/Vout Ctrl/vout_ctrl ==
  ixi_tilde : Inport
  0.14<x<0.45 : Saturate  UpperLimit=0.45  LowerLimit=0.14  OutDataTypeStr=double
  1/Ti : Gain  Gain=kp_v_zcs  ParamDataTypeStr=double  OutDataTypeStr=double  SaturateOnIntegerOverflow=on
  Sum1 : Sum  Inputs=+++  SaturateOnIntegerOverflow=on
  Sum4 : Sum  Inputs=-+  SaturateOnIntegerOverflow=on
  Unit Delay4 : UnitDelay  SampleTime=ts
  kp2 : Gain  Gain=ki_v_zcs*ts  ParamDataTypeStr=double  OutDataTypeStr=double  SaturateOnIntegerOverflow=on
  ctrlv_out : Outport
  wires:
  ixi_tilde/1 -> 1/Ti/1, kp2/1
  kp2/1 -> Sum1/2
  Sum4/1 -> Unit Delay4/1
  1/Ti/1 -> Sum1/1, Sum4/1
  Sum1/1 -> 0.14<x<0.45/1
  Unit Delay4/1 -> Sum1/3
  0.14<x<0.45/1 -> ctrlv_out/1, Sum4/2

== matlab function cll_zcs_ver_v/grid/grid_emulator/grid_emulator/voltage_reference/xieta2alphabeta_pos ==
  data: xi input; alpha output; eta input; gamma input; beta output
function [alpha,beta] = xieta2alphabeta_pos(xi,eta,gamma)

    alpha  =  xi*cos(gamma) - eta*sin(gamma);
    beta = xi*sin(gamma) + eta*cos(gamma);

end

== matlab function cll_zcs_ver_v/hs_compensation/magnitude_500Hz_harmonic_detection/kalman_observer ==
  data: y input; h1_hat output; w input; Ts input; q1 input; q2 input; r input; h2_hat output
function [h1_hat, h2_hat]   = KFO(y,w,Ts,q1,q2,r)

    persistent   x1_po x2_po p11_po p12_po p21_po p22_po

    if isempty(x1_po)
        x1_po = 0;
        x2_po = 0;
        p11_po = 0;
        p12_po = 0;
        p21_po = 0;
        p22_po = 0;        
    end
    
    a11 = cos(w*Ts);
    a12 = sin(w*Ts);
    a21 = -sin(w*Ts);
    a22 = cos(w*Ts);
    
    x1_pr = a11*x1_po + a12*x2_po;
    x2_pr = a21*x1_po + a22*x2_po;
    
    p11_pr = q1 + a11*(a11*p11_po+a12*p21_po) + a12*(a11*p12_po+a12*p22_po);
    p12_pr = a21*(a11*p11_po+a12*p21_po) + a22*(a11*p12_po+a12*p22_po);
    p21_pr = a11*(a21*p11_po+a22*p21_po) + a12*(a21*p12_po+a22*p22_po);
    p22_pr = q2 + a21*(a21*p11_po+a22*p21_po) + a22*(a21*p12_po+a22*p22_po);
    
    l1 = p11_pr/(p11_pr + r);
    l2 = p21_pr/(p11_pr + r);
    
    x1_po = x1_pr + l1*(y-x1_pr);
    x2_po = x2_pr + l2*(y-x1_pr);
    
    p11_po = (1-l1)*p11_pr;
    p12_po = (1-l1)*p12_pr;
    p21_po = p21_pr-l2*p11_pr;
    p22_po = p22_pr-l2*p12_pr;
    
    h1_hat = x1_pr;
    h2_hat = x2_pr;
end

== matlab function cll_zcs_ver_v/hs_compensation/magnitude_700Hz_harmonic_detection/double_integrator_observer/bounder1 ==
  data: u input; y output
function y = bounder(u)
    
    u = -pi + mod(u+3*pi,2*pi);
    
    y = u;
end

== matlab function cll_zcs_ver_v/hs_compensation/magnitude_700Hz_harmonic_detection/double_integrator_observer/bounder2 ==
  data: u input; y output
function y = bounder(u)
    
    u = -pi + mod(u+3*pi,2*pi);
    
    y = u;
end

== matlab function cll_zcs_ver_v/hs_compensation/magnitude_100Hz_harmonic_detection/double_integrator_observer/bounder1 ==
  data: u input; y output
function y = bounder(u)
    
    u = -pi + mod(u+3*pi,2*pi);
    
    y = u;
end

== matlab function cll_zcs_ver_v/hs_compensation/magnitude_100Hz_harmonic_detection/double_integrator_observer/bounder2 ==
  data: u input; y output
function y = bounder(u)
    
    u = -pi + mod(u+3*pi,2*pi);
    
    y = u;
end

== matlab function cll_zcs_ver_v/hs_compensation/magnitude_100Hz_harmonic_detection/kalman_observer ==
  data: y input; h1_hat output; w input; Ts input; q1 input; q2 input; r input; h2_hat output
function [h1_hat, h2_hat]   = KFO(y,w,Ts,q1,q2,r)

    persistent   x1_po x2_po p11_po p12_po p21_po p22_po

    if isempty(x1_po)
        x1_po = 0;
        x2_po = 0;
        p11_po = 0;
        p12_po = 0;
        p21_po = 0;
        p22_po = 0;        
    end
    
    a11 = cos(w*Ts);
    a12 = sin(w*Ts);
    a21 = -sin(w*Ts);
    a22 = cos(w*Ts);
    
    x1_pr = a11*x1_po + a12*x2_po;
    x2_pr = a21*x1_po + a22*x2_po;
    
    p11_pr = q1 + a11*(a11*p11_po+a12*p21_po) + a12*(a11*p12_po+a12*p22_po);
    p12_pr = a21*(a11*p11_po+a12*p21_po) + a22*(a11*p12_po+a12*p22_po);
    p21_pr = a11*(a21*p11_po+a22*p21_po) + a12*(a21*p12_po+a22*p22_po);
    p22_pr = q2 + a21*(a21*p11_po+a22*p21_po) + a22*(a21*p12_po+a22*p22_po);
    
    l1 = p11_pr/(p11_pr + r);
    l2 = p21_pr/(p11_pr + r);
    
    x1_po = x1_pr + l1*(y-x1_pr);
    x2_po = x2_pr + l2*(y-x1_pr);
    
    p11_po = (1-l1)*p11_pr;
    p12_po = (1-l1)*p12_pr;
    p21_po = p21_pr-l2*p11_pr;
    p22_po = p22_pr-l2*p12_pr;
    
    h1_hat = x1_pr;
    h2_hat = x2_pr;
end

== matlab function cll_zcs_ver_v/vi_ctrl/modulator/MATLAB Function ==
  data: in input; out output; tc input
function out = triangle(in,tc)

persistent y k

if isempty(y)
    y = 0;
    k = 1;
end

if y > 1
    k = -1;
    y = y + 4*k * in * tc;
elseif y < -1
    k = 1;
    y = y + 4*k * in * tc;
else
    y = y + 4*k * in * tc;
end
out = y;

== matlab function cll_zcs_ver_v/hs_compensation/magnitude_600Hz_harmonic_detection/double_integrator_observer/bounder1 ==
  data: u input; y output
function y = bounder(u)
    
    u = -pi + mod(u+3*pi,2*pi);
    
    y = u;
end

== matlab function cll_zcs_ver_v/hs_compensation/magnitude_600Hz_harmonic_detection/double_integrator_observer/bounder2 ==
  data: u input; y output
function y = bounder(u)
    
    u = -pi + mod(u+3*pi,2*pi);
    
    y = u;
end

== matlab function cll_zcs_ver_v/hs_compensation/magnitude_600Hz_harmonic_detection/kalman_observer ==
  data: y input; h1_hat output; w input; Ts input; q1 input; q2 input; r input; h2_hat output
function [h1_hat, h2_hat]   = KFO(y,w,Ts,q1,q2,r)

    persistent   x1_po x2_po p11_po p12_po p21_po p22_po

    if isempty(x1_po)
        x1_po = 0;
        x2_po = 0;
        p11_po = 0;
        p12_po = 0;
        p21_po = 0;
        p22_po = 0;        
    end
    
    a11 = cos(w*Ts);
    a12 = sin(w*Ts);
    a21 = -sin(w*Ts);
    a22 = cos(w*Ts);
    
    x1_pr = a11*x1_po + a12*x2_po;
    x2_pr = a21*x1_po + a22*x2_po;
    
    p11_pr = q1 + a11*(a11*p11_po+a12*p21_po) + a12*(a11*p12_po+a12*p22_po);
    p12_pr = a21*(a11*p11_po+a12*p21_po) + a22*(a11*p12_po+a12*p22_po);
    p21_pr = a11*(a21*p11_po+a22*p21_po) + a12*(a21*p12_po+a22*p22_po);
    p22_pr = q2 + a21*(a21*p11_po+a22*p21_po) + a22*(a21*p12_po+a22*p22_po);
    
    l1 = p11_pr/(p11_pr + r);
    l2 = p21_pr/(p11_pr + r);
    
    x1_po = x1_pr + l1*(y-x1_pr);
    x2_po = x2_pr + l2*(y-x1_pr);
    
    p11_po = (1-l1)*p11_pr;
    p12_po = (1-l1)*p12_pr;
    p21_po = p21_pr-l2*p11_pr;
    p22_po = p22_pr-l2*p12_pr;
    
    h1_hat = x1_pr;
    h2_hat = x2_pr;
end

== matlab function cll_zcs_ver_v/hs_compensation/magnitude_400Hz_harmonic_detection/double_integrator_observer/bounder1 ==
  data: u input; y output
function y = bounder(u)
    
    u = -pi + mod(u+3*pi,2*pi);
    
    y = u;
end

== matlab function cll_zcs_ver_v/hs_compensation/magnitude_400Hz_harmonic_detection/double_integrator_observer/bounder2 ==
  data: u input; y output
function y = bounder(u)
    
    u = -pi + mod(u+3*pi,2*pi);
    
    y = u;
end

== matlab function cll_zcs_ver_v/hs_compensation/magnitude_200Hz_harmonic_detection/double_integrator_observer/bounder1 ==
  data: u input; y output
function y = bounder(u)
    
    u = -pi + mod(u+3*pi,2*pi);
    
    y = u;
end

== matlab function cll_zcs_ver_v/hs_compensation/magnitude_200Hz_harmonic_detection/double_integrator_observer/bounder2 ==
  data: u input; y output
function y = bounder(u)
    
    u = -pi + mod(u+3*pi,2*pi);
    
    y = u;
end

== matlab function cll_zcs_ver_v/hs_compensation/magnitude_200Hz_harmonic_detection/kalman_observer ==
  data: y input; h1_hat output; w input; Ts input; q1 input; q2 input; r input; h2_hat output
function [h1_hat, h2_hat]   = KFO(y,w,Ts,q1,q2,r)

    persistent   x1_po x2_po p11_po p12_po p21_po p22_po

    if isempty(x1_po)
        x1_po = 0;
        x2_po = 0;
        p11_po = 0;
        p12_po = 0;
        p21_po = 0;
        p22_po = 0;        
    end
    
    a11 = cos(w*Ts);
    a12 = sin(w*Ts);
    a21 = -sin(w*Ts);
    a22 = cos(w*Ts);
    
    x1_pr = a11*x1_po + a12*x2_po;
    x2_pr = a21*x1_po + a22*x2_po;
    
    p11_pr = q1 + a11*(a11*p11_po+a12*p21_po) + a12*(a11*p12_po+a12*p22_po);
    p12_pr = a21*(a11*p11_po+a12*p21_po) + a22*(a11*p12_po+a12*p22_po);
    p21_pr = a11*(a21*p11_po+a22*p21_po) + a12*(a21*p12_po+a22*p22_po);
    p22_pr = q2 + a21*(a21*p11_po+a22*p21_po) + a22*(a21*p12_po+a22*p22_po);
    
    l1 = p11_pr/(p11_pr + r);
    l2 = p21_pr/(p11_pr + r);
    
    x1_po = x1_pr + l1*(y-x1_pr);
    x2_po = x2_pr + l2*(y-x1_pr);
    
    p11_po = (1-l1)*p11_pr;
    p12_po = (1-l1)*p12_pr;
    p21_po = p21_pr-l2*p11_pr;
    p22_po = p22_pr-l2*p12_pr;
    
    h1_hat = x1_pr;
    h2_hat = x2_pr;
end

== matlab function cll_zcs_ver_v/hs_compensation/magnitude_400Hz_harmonic_detection/kalman_observer ==
  data: y input; h1_hat output; w input; Ts input; q1 input; q2 input; r input; h2_hat output
function [h1_hat, h2_hat]   = KFO(y,w,Ts,q1,q2,r)

    persistent   x1_po x2_po p11_po p12_po p21_po p22_po

    if isempty(x1_po)
        x1_po = 0;
        x2_po = 0;
        p11_po = 0;
        p12_po = 0;
        p21_po = 0;
        p22_po = 0;        
    end
    
    a11 = cos(w*Ts);
    a12 = sin(w*Ts);
    a21 = -sin(w*Ts);
    a22 = cos(w*Ts);
    
    x1_pr = a11*x1_po + a12*x2_po;
    x2_pr = a21*x1_po + a22*x2_po;
    
    p11_pr = q1 + a11*(a11*p11_po+a12*p21_po) + a12*(a11*p12_po+a12*p22_po);
    p12_pr = a21*(a11*p11_po+a12*p21_po) + a22*(a11*p12_po+a12*p22_po);
    p21_pr = a11*(a21*p11_po+a22*p21_po) + a12*(a21*p12_po+a22*p22_po);
    p22_pr = q2 + a21*(a21*p11_po+a22*p21_po) + a22*(a21*p12_po+a22*p22_po);
    
    l1 = p11_pr/(p11_pr + r);
    l2 = p21_pr/(p11_pr + r);
    
    x1_po = x1_pr + l1*(y-x1_pr);
    x2_po = x2_pr + l2*(y-x1_pr);
    
    p11_po = (1-l1)*p11_pr;
    p12_po = (1-l1)*p12_pr;
    p21_po = p21_pr-l2*p11_pr;
    p22_po = p22_pr-l2*p12_pr;
    
    h1_hat = x1_pr;
    h2_hat = x2_pr;
end

== matlab function cll_zcs_ver_v/hs_compensation/magnitude_700Hz_harmonic_detection/kalman_observer ==
  data: y input; h1_hat output; w input; Ts input; q1 input; q2 input; r input; h2_hat output
function [h1_hat, h2_hat]   = KFO(y,w,Ts,q1,q2,r)

    persistent   x1_po x2_po p11_po p12_po p21_po p22_po

    if isempty(x1_po)
        x1_po = 0;
        x2_po = 0;
        p11_po = 0;
        p12_po = 0;
        p21_po = 0;
        p22_po = 0;        
    end
    
    a11 = cos(w*Ts);
    a12 = sin(w*Ts);
    a21 = -sin(w*Ts);
    a22 = cos(w*Ts);
    
    x1_pr = a11*x1_po + a12*x2_po;
    x2_pr = a21*x1_po + a22*x2_po;
    
    p11_pr = q1 + a11*(a11*p11_po+a12*p21_po) + a12*(a11*p12_po+a12*p22_po);
    p12_pr = a21*(a11*p11_po+a12*p21_po) + a22*(a11*p12_po+a12*p22_po);
    p21_pr = a11*(a21*p11_po+a22*p21_po) + a12*(a21*p12_po+a22*p22_po);
    p22_pr = q2 + a21*(a21*p11_po+a22*p21_po) + a22*(a21*p12_po+a22*p22_po);
    
    l1 = p11_pr/(p11_pr + r);
    l2 = p21_pr/(p11_pr + r);
    
    x1_po = x1_pr + l1*(y-x1_pr);
    x2_po = x2_pr + l2*(y-x1_pr);
    
    p11_po = (1-l1)*p11_pr;
    p12_po = (1-l1)*p12_pr;
    p21_po = p21_pr-l2*p11_pr;
    p22_po = p22_pr-l2*p12_pr;
    
    h1_hat = x1_pr;
    h2_hat = x2_pr;
end

== matlab function cll_zcs_ver_v/PLL/pll_stageA/mormalization_and_transformation/abc2alphabeta ==
  data: a input; alpha output; b input; c input; beta output
function [alpha,beta] = abc2alphabeta(a,b,c)

alpha = 2/3*(a - 1/2*b - 1/2*c);
beta  = 1/sqrt(3)*(b - c);

end

== matlab function cll_zcs_ver_v/PLL/pll_stageA/sequences/ddsrf/alphabeta2xieta_neg ==
  data: alpha input; xi output; beta input; gamma input; eta output
function [xi,eta] = alphabeta2xieta_neg(alpha,beta,gamma)

    xi  = alpha*cos(gamma) - beta*sin(gamma);
    eta = alpha*sin(gamma) + beta*cos(gamma);

end

== matlab function cll_zcs_ver_v/PLL/pll_stageA/sequences/ddsrf/alphabeta2xieta_neg1 ==
  data: alpha input; xi output; beta input; gamma input; eta output
function [xi,eta] = alphabeta2xieta_neg(alpha,beta,gamma)

    xi  = alpha*cos(gamma) - beta*sin(gamma);
    eta = alpha*sin(gamma) + beta*cos(gamma);

end

== matlab function cll_zcs_ver_v/PLL/pll_stageA/sequences/ddsrf/alphabeta2xieta_pos ==
  data: alpha input; xi output; beta input; gamma input; eta output
function [xi,eta] = alphabeta2xieta_pos(alpha,beta,gamma)

    xi  =  alpha*cos(gamma) + beta*sin(gamma);
    eta = -alpha*sin(gamma) + beta*cos(gamma);

end

== matlab function cll_zcs_ver_v/PLL/pll_stageA/sequences/ddsrf/alphabeta2xieta_pos1 ==
  data: alpha input; xi output; beta input; gamma input; eta output
function [xi,eta] = alphabeta2xieta_pos(alpha,beta,gamma)

    xi  =  alpha*cos(gamma) + beta*sin(gamma);
    eta = -alpha*sin(gamma) + beta*cos(gamma);

end

== matlab function cll_zcs_ver_v/PLL/pll_stageA/sequences/ddsrf/bounder2 ==
  data: u input; y output
function y = bounder(u)
    
    u = -pi + mod(u+3*pi,2*pi);
    
    y = u;
end

== matlab function cll_zcs_ver_v/grid/grid_emulator/grid_emulator/phase_gen/bounder1 ==
  data: u input; y output
function y = bounder(u)
    
    u = -pi + mod(u+3*pi,2*pi);
    
    y = u;
end

== matlab function cll_zcs_ver_v/PLL/pll_stageB/bounder1 ==
  data: u input; y output
function y = bounder(u)
    
    u = -pi + mod(u+3*pi,2*pi);
    
    y = u;
end

== matlab function cll_zcs_ver_v/PLL/pll_stageB/double_integrator_observer/bounder1 ==
  data: u input; y output
function y = bounder(u)
    
    u = -pi + mod(u+3*pi,2*pi);
    
    y = u;
end

== matlab function cll_zcs_ver_v/PLL/pll_stageB/double_integrator_observer/bounder2 ==
  data: u input; y output
function y = bounder(u)
    
    u = -pi + mod(u+3*pi,2*pi);
    
    y = u;
end

== matlab function cll_zcs_ver_v/hs_compensation/magnitude_300Hz_harmonic_detection/kalman_observer ==
  data: y input; h1_hat output; w input; Ts input; q1 input; q2 input; r input; h2_hat output
function [h1_hat, h2_hat]   = KFO(y,w,Ts,q1,q2,r)

    persistent   x1_po x2_po p11_po p12_po p21_po p22_po

    if isempty(x1_po)
        x1_po = 0;
        x2_po = 0;
        p11_po = 0;
        p12_po = 0;
        p21_po = 0;
        p22_po = 0;        
    end
    
    a11 = cos(w*Ts);
    a12 = sin(w*Ts);
    a21 = -sin(w*Ts);
    a22 = cos(w*Ts);
    
    x1_pr = a11*x1_po + a12*x2_po;
    x2_pr = a21*x1_po + a22*x2_po;
    
    p11_pr = q1 + a11*(a11*p11_po+a12*p21_po) + a12*(a11*p12_po+a12*p22_po);
    p12_pr = a21*(a11*p11_po+a12*p21_po) + a22*(a11*p12_po+a12*p22_po);
    p21_pr = a11*(a21*p11_po+a22*p21_po) + a12*(a21*p12_po+a22*p22_po);
    p22_pr = q2 + a21*(a21*p11_po+a22*p21_po) + a22*(a21*p12_po+a22*p22_po);
    
    l1 = p11_pr/(p11_pr + r);
    l2 = p21_pr/(p11_pr + r);
    
    x1_po = x1_pr + l1*(y-x1_pr);
    x2_po = x2_pr + l2*(y-x1_pr);
    
    p11_po = (1-l1)*p11_pr;
    p12_po = (1-l1)*p12_pr;
    p21_po = p21_pr-l2*p11_pr;
    p22_po = p22_pr-l2*p12_pr;
    
    h1_hat = x1_pr;
    h2_hat = x2_pr;
end

== matlab function cll_zcs_ver_v/hs_compensation/magnitude_300Hz_harmonic_detection/double_integrator_observer/bounder1 ==
  data: u input; y output
function y = bounder(u)
    
    u = -pi + mod(u+3*pi,2*pi);
    
    y = u;
end

== matlab function cll_zcs_ver_v/hs_compensation/magnitude_300Hz_harmonic_detection/double_integrator_observer/bounder2 ==
  data: u input; y output
function y = bounder(u)
    
    u = -pi + mod(u+3*pi,2*pi);
    
    y = u;
end

== matlab function cll_zcs_ver_v/hs_compensation/magnitude_500Hz_harmonic_detection/double_integrator_observer/bounder1 ==
  data: u input; y output
function y = bounder(u)
    
    u = -pi + mod(u+3*pi,2*pi);
    
    y = u;
end

== matlab function cll_zcs_ver_v/hs_compensation/magnitude_500Hz_harmonic_detection/double_integrator_observer/bounder2 ==
  data: u input; y output
function y = bounder(u)
    
    u = -pi + mod(u+3*pi,2*pi);
    
    y = u;
end

== matlab function cll_zcs_ver_v/grid/grid_emulator/grid_emulator/voltage_reference/alphabeta2abc ==
  data: alpha input; a output; beta input; b output; c output
function [a,b,c] = alphabeta2abc(alpha,beta)

    a  =  alpha;
    b  =  -0.5*alpha + sqrt(3)/2*beta;
    c  =  -0.5*alpha - sqrt(3)/2*beta;
end

== matlab function cll_zcs_ver_v/grid/grid_emulator/grid_emulator/voltage_reference/xieta2alphabeta_neg ==
  data: xi input; alpha output; eta input; gamma input; beta output
function [alpha,beta] = xieta2alphabeta_neg(xi,eta,gamma)

    alpha  =  xi*cos(gamma) + eta*sin(gamma);
    beta = -xi*sin(gamma) + eta*cos(gamma);

end
